simulink model "os1"  (R2026b)
settings: Solver=VariableStepAuto  StopTime=Tsim  MaxStep=0.01
undefined symbols (not defined in the file): az, t_skok
settings Model: Creator=Jakub  LastModifiedBy=Jakub

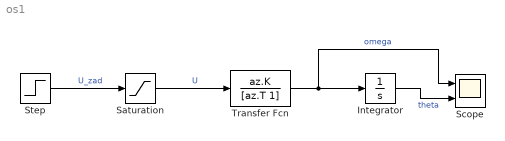
== system os1 ==
  Integrator : Integrator
  Saturation : Saturate  UpperLimit=az.Umax  LowerLimit=-az.Umax
  Scope : Scope  NumInputPorts=2
      settings: ActiveDisplayYMinimum=-2.0292963402588966  ActiveDisplayYMaximum=7.08699785234238
  Step : Step  Time=t_skok  FinalValue=U_skok  SampleTime=0
  Transfer Fcn : TransferFcn  Numerator=az.K  Denominator=[az.T 1]
  wires:
  Step/1 -> Saturation/1  "U_zad"
  Saturation/1 -> Transfer Fcn/1  "U"
  Transfer Fcn/1 -> Scope/1, Integrator/1  "omega"
  Integrator/1 -> Scope/2  "theta"
